simulink model "pid_anti_windup_clamping_ver2"  (R2026b)
settings: Solver=ode4  StopTime=30  FixedStep=0.05
libraries: simulink x2
settings Model: Creator=ZAID  LastModifiedBy=ZAID

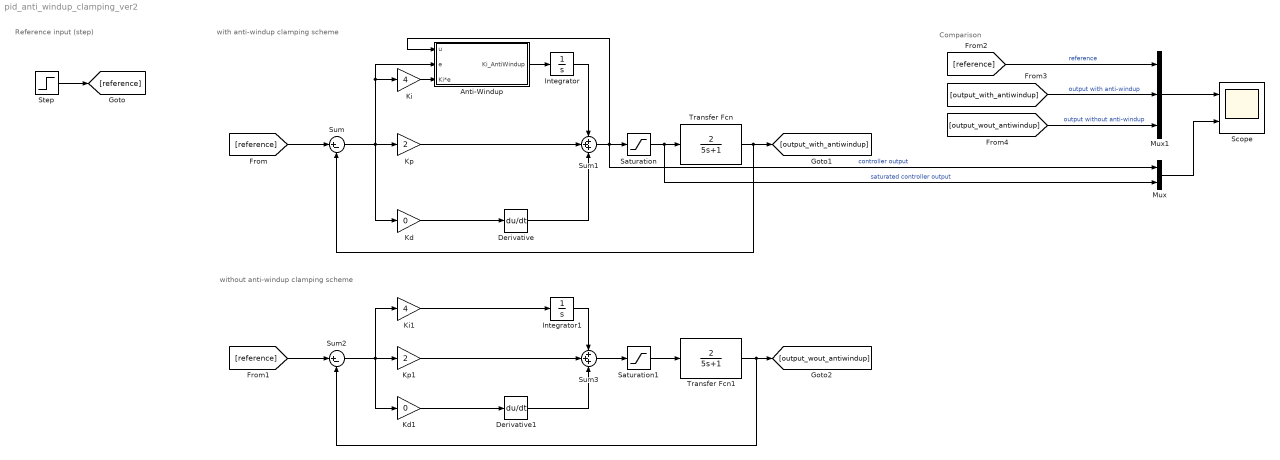
== system pid_anti_windup_clamping_ver2 ==
  note: Comparison
  note: Reference input (step)
  note: without anti-windup clamping scheme
  note: with anti-windup clamping scheme
  Anti-Windup : Subsystem
  Derivative : Derivative
  Derivative1 : Derivative
  Integrator : Integrator
  Integrator1 : Integrator
  Kd : Gain  Gain=0
  Kd1 : Gain  Gain=0
  Ki : Gain  Gain=4
  Ki1 : Gain  Gain=4
  Kp : Gain  Gain=2
  Kp1 : Gain  Gain=2
  Mux : Mux  Inputs=2
  Mux1 : Mux  Inputs=3
  Saturation : Saturate  UpperLimit=10  LowerLimit=-10
      settings: AttributesFormatString=|
      | u_max = %<UpperLimit>
      | u_min = %<LowerLimit>
  Saturation1 : Saturate  UpperLimit=10  LowerLimit=-10
      settings: AttributesFormatString=|
      | u_max = %<UpperLimit>
      | u_min = %<LowerLimit>
  Scope : Scope  NumInputPorts=2
      settings: ActiveDisplayYMinimum=-2.4389081814821214  ActiveDisplayYMaximum=21.950173633339098
  Step : Step  FinalValue=15  SampleTime=0
  Sum : Sum  Inputs=|+-
  Sum1 : Sum  Inputs=+++
  Sum2 : Sum  Inputs=|+-
  Sum3 : Sum  Inputs=+++
  Transfer Fcn : TransferFcn  Numerator=2  Denominator=[5 1]
  Transfer Fcn1 : TransferFcn  Numerator=2  Denominator=[5 1]
  wires:
  [output_with_antiwindup] -> Mux1/2  "output with anti-windup"
  Saturation1/1 -> Transfer Fcn1/1
  Kp1/1 -> Sum3/2
  [reference] -> Sum/1
  Sum2/1 -> Kp1/1, Kd1/1, Ki1/1
  Derivative/1 -> Sum1/3
  Kd/1 -> Derivative/1
  Step/1 -> [reference]
  [reference] -> Mux1/1  "reference"
  Sum1/1 -> Anti-Windup/1(u), Mux/1, Saturation/1  "controller output"
  Kp/1 -> Sum1/2
  Anti-Windup/1(Ki_AntiWindup) -> Integrator/1
  Integrator1/1 -> Sum3/1
  Transfer Fcn1/1 -> Sum2/2, [output_wout_antiwindup]
  Integrator/1 -> Sum1/1
  Ki1/1 -> Integrator1/1
  Sum/1 -> Anti-Windup/2(e), Ki/1, Kd/1, Kp/1
  Transfer Fcn/1 -> [output_with_antiwindup], Sum/2
  Ki/1 -> Anti-Windup/3(Ki*e)
  Saturation/1 -> Mux/2, Transfer Fcn/1  "saturated controller output"
  Derivative1/1 -> Sum3/3
  [output_wout_antiwindup] -> Mux1/3  "output without anti-windup"
  [reference] -> Sum2/1
  Kd1/1 -> Derivative1/1
  Sum3/1 -> Saturation1/1
  Mux1/1 -> Scope/1
  Mux/1 -> Scope/2

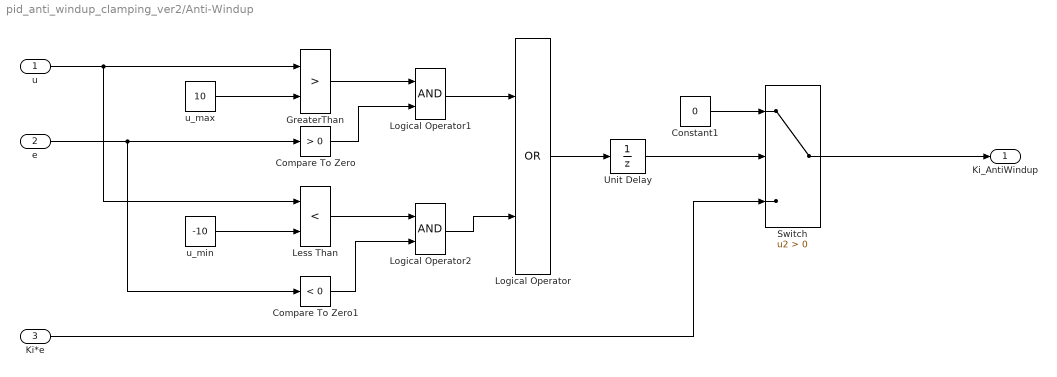
== system pid_anti_windup_clamping_ver2/Anti-Windup ==
  u : Inport
  e : Inport  Port=2
  Ki*e : Inport  Port=3
  Compare To Zero : simulink/Logic and Bit Operations/Compare To Zero  relop=>  OutDataTypeStr=boolean
  Compare To Zero1 : simulink/Logic and Bit Operations/Compare To Zero  relop=<  OutDataTypeStr=boolean
  Constant1 : Constant  Value=0
  GreaterThan : RelationalOperator  Operator=>  OutDataTypeStr=boolean  RndMeth=Simplest  InputSameDT=off
  Less Than : RelationalOperator  Operator=<  OutDataTypeStr=boolean  RndMeth=Simplest  InputSameDT=off
  Logical Operator : Logic  Operator=OR  AllPortsSameDT=off  OutDataTypeStr=boolean
  Logical Operator1 : Logic  AllPortsSameDT=off  OutDataTypeStr=boolean
  Logical Operator2 : Logic  AllPortsSameDT=off  OutDataTypeStr=boolean
  Switch : Switch  Criteria=u2 > Threshold  SaturateOnIntegerOverflow=off  InputSameDT=off
  Unit Delay : UnitDelay  SampleTime=-1
  u_max : Constant  Value=10
  u_min : Constant  Value=-10
  Ki_AntiWindup : Outport
  wires:
  u/1 -> Less Than/1, GreaterThan/1
  Switch/1 -> Ki_AntiWindup/1
  u_min/1 -> Less Than/2
  u_max/1 -> GreaterThan/2
  Logical Operator/1 -> Unit Delay/1
  Ki*e/1 -> Switch/3
  Constant1/1 -> Switch/1
  GreaterThan/1 -> Logical Operator1/1
  e/1 -> Compare To Zero1/1, Compare To Zero/1
  Compare To Zero/1 -> Logical Operator1/2
  Logical Operator1/1 -> Logical Operator/1
  Less Than/1 -> Logical Operator2/1
  Logical Operator2/1 -> Logical Operator/2
  Compare To Zero1/1 -> Logical Operator2/2
  Unit Delay/1 -> Switch/2
